simulink model "Model_A"  (R2024b)
settings: Solver=ode15s  StartTime=0.0  StopTime=3  MaxStep=0.001  RelTol=9.9999999999999995e-08  AbsTol=1.0000000000000001e-09
PostLoadFcn:
  | addpath(fileparts(get_param(bdroot,'FileName')));
InitFcn:
  | Model_A_initialize(bdroot);
model workspace (MAT data in the model file):
  ic.x0 = [0.0487207667186; 0; 1.03532101344; 2.70319926687e-24]
  ic.V0 = 0.998847335682-0.048i
  ic.Vnom = 1
  ic.network = [0.998847335682; -0.048; 1; 1; 0.414093240727; 1.04542083745; 0.30480276799; 39666.4759309; 0; 1.22124532709e-15; 12.929734979; 0]
  ic.residual = 1.21569421196e-14
  ic.eigenvalues = [-0.599279843882+14.9008401777i; -0.599279843882-14.9008401777i; -5.25574712927+0i; -62.8318530718+0i]
  networkParameters = [0.1; 0; 0.24; 1.2; 0.3; 1; 0; 0.01; 0; 1; 1]
  p.baseMVA = 100
  p.freq = 60
  p.M = 5.0224
  p.D = 6
  p.K = 12
  p.Dq = 60
  p.xe = 0.1
  p.xL1 = 0
  p.xL2 = 0.24
  p.PL = 1.2
  p.QL = 0.3
  p.VS = 1
  p.thetaS = 0
  p.Pref = 1
  p.Eref = 1.03532101344
  p.Qref = 0.414093240727
  p.Ithresh = 1.1
  p.Imax = 1.5
  p.SigmaXR = 5
  p.Vmax = 1
  p.KVI = 0.283333333333
  p.omegaVI = 62.8318530718
  p.xvmax = 0.566666666667
  p.faultEnabled = 1
  p.tFault = 0.1
  p.tClear = 0.18
  p.Rf = 0.01
  p.Xf = 0
  p.faultLoadToZ = 1
  p.Vswitch = 1
  p.tStop = 3
  p.solver = 'ode15s'
  p.maxStep = 0.001
  p.relTol = 1e-07
  p.absTol = 1e-09
  p.initTol = 1e-09
  p.residualTol = 1e-07
  p.showFigures = 0
  p.saveResults = 0
  p.outputDir = 'D:\matlab\威\威-1304-售后-200-10.20\调试副本_20261019\ModelA\Model_A_results'
values from neighbouring files (symbols this model uses):
  ic = Model_A_initial_state(p)    [Model_A_initialize.m]
  p = Model_A_parameters()    [Model_A_initialize.m]
settings Model: Creator=Administrator  LastModifiedBy=Administrator
settings DataIOCC: SaveOutput=off  SignalLogging=off

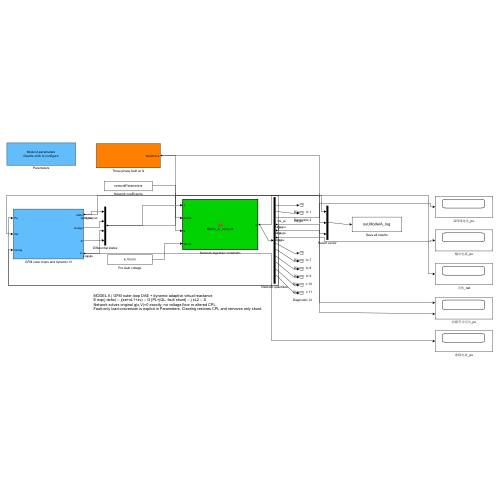
[thumbnail: Simulink's stored preview of the top-level diagram]
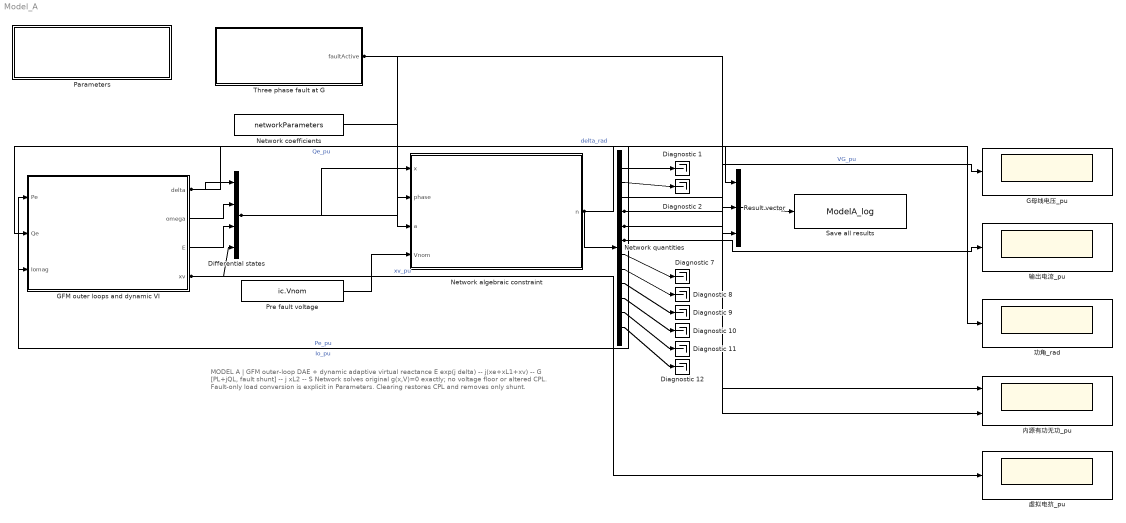
== system Model_A ==
  note: MODEL A | GFM outer-loop DAE + dynamic adaptive virtual reactance
      | E exp(j delta) -- j(xe+xL1+xv) -- G [PL+jQL, fault shunt] -- j xL2 -- S
      | Network solves original g(x,V)=0 exactly; no voltage floor or altered CPL.
      | Fault-only load conversion is explicit in Parameters. Clearing restores CPL and removes only shunt.
  Diagnostic {1..2,7..12} (8 alike) : Terminator
  Differential states : Mux
  GFM outer loops and dynamic VI : Subsystem
  G母线电压_pu : Scope
  Network algebraic constraint : MATLAB Function  TreatAsAtomicUnit=on
  Network coefficients : Constant  Value=networkParameters
  Network quantities : Demux  Outputs=12
  Parameters : Subsystem  mask{baseMVA=100, freq=60, M=5.0224000000000002, D=6, K=12, Dq=60, xe=0.10000000000000001, xL1=0, xL2=0.23999999999999999, PL=1.2, QL=0.29999999999999999, VS=1, thetaS=0, Pref=1, Eref=1.0353210134405997, Qref=0.41409324072705855, Ithresh=1.1000000000000001, Imax=1.5, SigmaXR=5, Vmax=1, KVI=0.28333333333333344, omegaVI=62.831853071795862, xvmax=0.56666666666666676, faultEnabled=1, tFault=0.10000000000000001, tClear=0.17999999999999999, Rf=0.01, Xf=0, faultLoadToZ=1, Vswitch=1, tStop=3, maxStep=0.001, relTol=9.9999999999999995e-08, absTol=1.0000000000000001e-09, initTol=1.0000000000000001e-09, residualTol=9.9999999999999995e-08, solverName=ode15s}
      mask prompts: baseMVA "Base power (MVA)"; freq "Nominal frequency (Hz)"; M "Virtual inertia M"; D "Active damping D"; K "Voltage integral K"; Dq "Q-V droop Dq"; xe "Converter reactance xe (pu)"; xL1 "Line xL1 (pu), included in original Xe"; xL2 "Line G-S xL2 (pu)"; PL "Load PL (pu)"; QL "Load QL (pu)"; VS "Infinite-bus voltage (pu)"; thetaS "Infinite-bus angle (rad)"; Pref "Active reference Pref (pu)"; Eref "Internal voltage reference Eref (pu)"; Qref "Internal reactive reference Qref (pu)"; Ithresh "VI threshold Ithresh (pu)"; Imax "Design current Imax (pu), not a hard limiter"; SigmaXR "VI design X/R ratio"; Vmax "Design maximum voltage difference (pu)"; KVI "VI gain KVI"; omegaVI "VI response omegaVI (rad/s)"; xvmax "Analysis bound xvmax (pu), no saturation"; faultEnabled "Fault enabled (0 or 1)"; tFault "Fault inception time (s)"; tClear "Fault clearing time (s)"; Rf "Fault resistance Rf (pu)"; Xf "Fault reactance Xf (pu)"; faultLoadToZ "Fault-only CP to Z conversion (0 or 1)"; Vswitch "Voltage switching threshold (pu)"; tStop "Stop time (s)"; maxStep "Maximum solver step (s)"; relTol "Relative tolerance"; absTol "Absolute tolerance"; initTol "Initialization tolerance"; residualTol "Algebraic residual tolerance"; solverName "Solver"
      mask help: Model A: paper outer-loop DAE with adaptive virtual reactance. Modify these values, Apply, then Run. Initialization recalculates the SEP. xe+xL1 equals original code Xe. xvmax is an analysis bound, not a limiter.
      mask TypeOptions solverName: ode15s | ode23t | ode23tb | ode45
      mask DialogControl tab1 Prompt: System and GFM
      mask DialogControl tab2 Prompt: Network and load
      mask DialogControl tab3 Prompt: Power references
      mask DialogControl tab4 Prompt: Virtual reactance
      mask DialogControl tab5 Prompt: Three-phase fault at G
      mask DialogControl tab6 Prompt: Simulation and diagnostics
      mask Display: disp('Model A parameters\nDouble-click to configure')
  Pre fault voltage : Constant  Value=ic.Vnom
  Result vector : Mux  Inputs=3
  Save all results : ToWorkspace  VariableName=ModelA_log  SaveFormat=Timeseries  SampleTime=-1
  Three phase fault at G : Subsystem
  内源有功无功_pu : Scope  NumInputPorts=2
  功角_rad : Scope
  虚拟电抗_pu : Scope
  输出电流_pu : Scope
  wires:
  Differential states/1 -> Network algebraic constraint/1(x), Result vector/1
  Three phase fault at G/1(faultActive) -> Network algebraic constraint/2(phase), Result vector/3
  Network coefficients/1 -> Network algebraic constraint/3(a)
  Pre fault voltage/1 -> Network algebraic constraint/4(Vnom)
  Network algebraic constraint/1(n) -> Network quantities/1, Result vector/2
  GFM outer loops and dynamic VI/1(delta) -> Differential states/1, 功角_rad/1  "delta_rad"
  GFM outer loops and dynamic VI/2(omega) -> Differential states/2
  GFM outer loops and dynamic VI/3(E) -> Differential states/3
  GFM outer loops and dynamic VI/4(xv) -> Differential states/4, 虚拟电抗_pu/1  "xv_pu"
  Network quantities/4 -> GFM outer loops and dynamic VI/1(Pe), 内源有功无功_pu/1  "Pe_pu"
  Network quantities/5 -> GFM outer loops and dynamic VI/2(Qe), 内源有功无功_pu/2  "Qe_pu"
  Network quantities/6 -> GFM outer loops and dynamic VI/3(Iomag), 输出电流_pu/1  "Io_pu"
  Result vector/1 -> Save all results/1
  Network quantities/3 -> G母线电压_pu/1  "VG_pu"
  Network quantities/1 -> Diagnostic 1/1
  Network quantities/2 -> Diagnostic 2/1
  Network quantities/7 -> Diagnostic 7/1
  Network quantities/8 -> Diagnostic 8/1
  Network quantities/9 -> Diagnostic 9/1
  Network quantities/10 -> Diagnostic 10/1
  Network quantities/11 -> Diagnostic 11/1
  Network quantities/12 -> Diagnostic 12/1

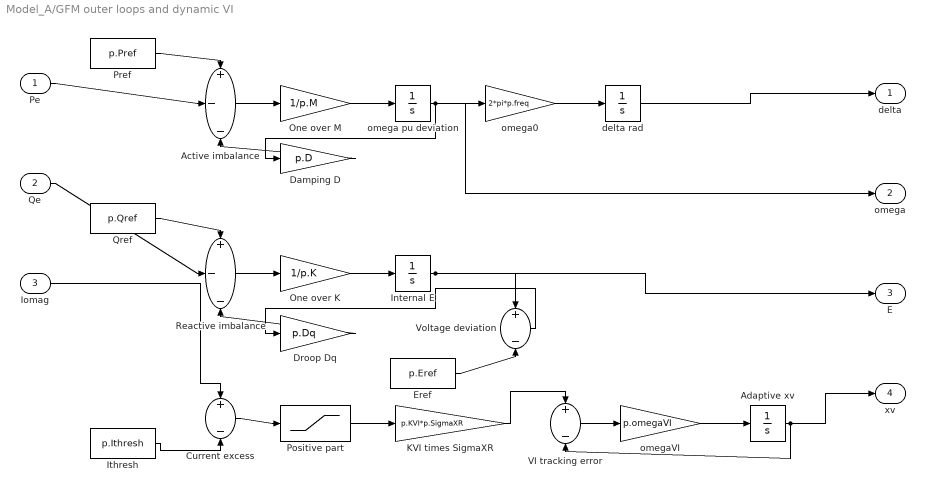
== system Model_A/GFM outer loops and dynamic VI ==
  Pe : Inport
  Qe : Inport  Port=2
  Iomag : Inport  Port=3
  Active imbalance : Sum  Inputs=+--
  Adaptive xv : Integrator  InitialCondition=ic.x0(4)
  Current excess : Sum  Inputs=+-
  Damping D : Gain  Gain=p.D
  Droop Dq : Gain  Gain=p.Dq
  Eref : Constant  Value=p.Eref
  Internal E : Integrator  InitialCondition=ic.x0(3)
  Ithresh : Constant  Value=p.Ithresh
  KVI times SigmaXR : Gain  Gain=p.KVI*p.SigmaXR
  One over K : Gain  Gain=1/p.K
  One over M : Gain  Gain=1/p.M
  Positive part : Saturate  UpperLimit=inf  LowerLimit=0
  Pref : Constant  Value=p.Pref
  Qref : Constant  Value=p.Qref
  Reactive imbalance : Sum  Inputs=+--
  VI tracking error : Sum  Inputs=+-
  Voltage deviation : Sum  Inputs=+-
  delta rad : Integrator  InitialCondition=ic.x0(1)
  omega pu deviation : Integrator  InitialCondition=ic.x0(2)
  omega0 : Gain  Gain=2*pi*p.freq
  omegaVI : Gain  Gain=p.omegaVI
  delta : Outport
  omega : Outport  Port=2
  E : Outport  Port=3
  xv : Outport  Port=4
  wires:
  Pref/1 -> Active imbalance/1
  Pe/1 -> Active imbalance/2
  Damping D/1 -> Active imbalance/3
  Active imbalance/1 -> One over M/1
  One over M/1 -> omega pu deviation/1
  omega pu deviation/1 -> Damping D/1, omega0/1, omega/1
  omega0/1 -> delta rad/1
  Qref/1 -> Reactive imbalance/1
  Qe/1 -> Reactive imbalance/2
  Droop Dq/1 -> Reactive imbalance/3
  Reactive imbalance/1 -> One over K/1
  One over K/1 -> Internal E/1
  Internal E/1 -> Voltage deviation/1, E/1
  Eref/1 -> Voltage deviation/2
  Voltage deviation/1 -> Droop Dq/1
  Iomag/1 -> Current excess/1
  Ithresh/1 -> Current excess/2
  Current excess/1 -> Positive part/1
  Positive part/1 -> KVI times SigmaXR/1
  KVI times SigmaXR/1 -> VI tracking error/1
  VI tracking error/1 -> omegaVI/1
  omegaVI/1 -> Adaptive xv/1
  Adaptive xv/1 -> VI tracking error/2, xv/1
  delta rad/1 -> delta/1

== system Model_A/Parameters ==

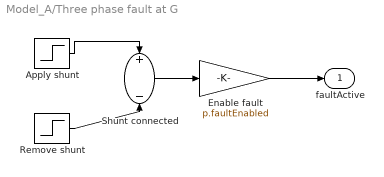
== system Model_A/Three phase fault at G ==
  Apply shunt : Step  Time=p.tFault  SampleTime=0
  Enable fault : Gain  Gain=p.faultEnabled
  Remove shunt : Step  Time=p.tClear  SampleTime=0
  Shunt connected : Sum  Inputs=+-
  faultActive : Outport
  wires:
  Apply shunt/1 -> Shunt connected/1
  Remove shunt/1 -> Shunt connected/2
  Shunt connected/1 -> Enable fault/1
  Enable fault/1 -> faultActive/1

== matlab function Model_A/Network algebraic constraint ==
  data: x input; n output; phase input; a input; Vnom input
function n = Model_A_network(x, phase, a, Vnom)
%#codegen
% EXACT algebraic solve of the paper's single-load-bus DAE, high-voltage
% component connected to the pre-fault SEP. No voltage floor/regularization.
% x=[delta; omega_pu_deviation; E; xv]
% a=[xe;xL1;xL2;PL;QL;VS;thetaS;Rf;Xf;faultLoadToZ;Vswitch]
% n=[Vr;Vi;|V|;Pe;Qe;|I|;Qbus;CP discriminant;loadZ;
%    |g|inf;sigma_min(dg/d[Vr,Vi]);xv_command_unused]
n = zeros(12,1);
X = a(1)+a(2)+x(4);
assert(X>0 && a(3)>0, 'Model_A: nonpositive equivalent reactance.');
Ei = x(3)*exp(1i*x(1));
Vs = a(6)*exp(1i*a(7));
Y = 1/(1i*X) + 1/(1i*a(3));
if phase == 1
    Y = Y + 1/complex(a(8),a(9));
end
A = Ei/(1i*X) + Vs/(1i*a(3));
S = complex(a(4),a(5));
aa = abs(Y)^2;
b = abs(A)^2-2*real(Y*S);
disc = b*b-4*aa*abs(S)^2;
cpExists = disc>=0 && b>0 && abs(A)>0;
Vcp = complex(0,0);
if cpExists
    u = (b+sqrt(disc))/(2*aa);
    Vcp = conj((Y*u+conj(S))/A);
end
loadZ = false;
V = Vcp;
if phase == 1 && a(10) ~= 0
    % The Z admittance uses the newly solved pre-fault voltage, as V0 in
    % runsimulation.m. Candidate selection solves the piecewise constraint
    % directly even when the fault CP equation has no real root.
    Vz = A/(Y+conj(S)/(Vnom*Vnom));
    if (~cpExists || abs(Vcp)<a(11)) && abs(Vz)<a(11)
        V = Vz;
        loadZ = true;
    end
end
assert(cpExists || loadZ, ...
 'Model_A_DAE_NO_REAL_SOLUTION: original algebraic constraint has no high-voltage real solution.');
assert(abs(V)>0, 'Model_A_DAE_ZERO_VOLTAGE: CPL voltage is zero.');
if loadZ
    Seff = S*abs(V)^2/(Vnom*Vnom);
else
    assert(disc>0, 'Model_A_DAE_SINGULAR: algebraic branches meet.');
    Seff = S;
end
I = (Ei-V)/(1i*X);
Sint = Ei*conj(I);
Sbus = V*conj(I);
% Original paper power-balance residual (negative sign is immaterial).
g = V*conj(A-Y*V)-Seff;
vr = real(V); vi = imag(V); G = real(Y); B = imag(Y);
% d/d[Vr,Vi] of [real(g);imag(g)], WITHOUT voltage perturbation.
J = [real(A)-2*G*vr, imag(A)-2*G*vi; ...
    -imag(A)+2*B*vr, real(A)+2*B*vi];
if loadZ
    J = J - 2/(Vnom*Vnom)*[a(4)*vr,a(4)*vi;a(5)*vr,a(5)*vi];
end
sv = svd(J);
n(1:11) = [vr;vi;abs(V);real(Sint);imag(Sint);abs(I); ...
    imag(Sbus);disc;double(loadZ);max(abs([real(g);imag(g)]));min(sv)];
end
